simulink model "dc_motor_plant"  (R2026a)
settings: Solver=ode4  StartTime=0  StopTime=5  FixedStep=0.00001
model workspace (MAT data in the model file):
  A = [-4  -0.2; 3.33333333333  -0.0333333333333]
  B = [2  0; 0  -33.3333333333]
  C = [0  1; 1  0]
  D = [0  0; 0  0]
  x0 = [0; 0]
settings Model: Creator=ievge  LastModifiedBy=ievge

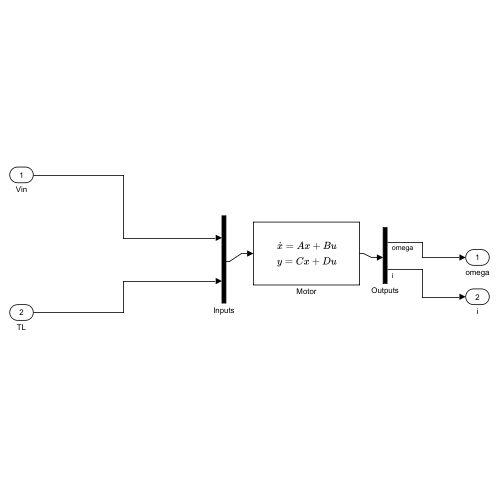
[thumbnail: Simulink's stored preview of the top-level diagram]
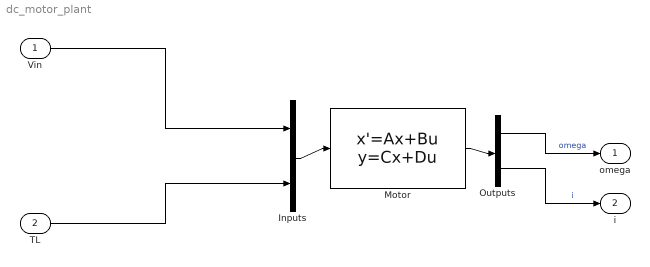
== system dc_motor_plant ==
  Vin : Inport  Unit=V
  TL : Inport  Port=2  Unit=N*m
  Inputs : Mux  Inputs=2
  Motor : StateSpace  A=A  B=B  C=C  D=D  InitialCondition=x0
  Outputs : Demux  Outputs=2
  omega : Outport  Unit=rad/s
  i : Outport  Port=2  Unit=A
  wires:
  Inputs/1 -> Motor/1
  Motor/1 -> Outputs/1
  TL/1 -> Inputs/2
  Outputs/1 -> omega/1  "omega"
  Outputs/2 -> i/1  "i"
  Vin/1 -> Inputs/1
